simulink model "SVPWM6kHz"  (R2025b)
settings: Solver=VariableStepAuto  StartTime=0.0  StopTime=2  MaxStep=1e-6  RelTol=1e-3  EnableMultiTasking=on
undefined symbols (not defined in the file): Down, SVPWM6kHz, Up
libraries: nesl_utility x11, ee_lib x7, fl_lib x6, peripheralslib x3, prociolib x3, slpidlib x2, eeTransforms x2, simulink x1, eeSinusoidalMeasurement x1
settings Model: ExtModeTrigDuration=8  Creator=18483  LastModifiedBy=18483
settings OptimizationCC: DefaultParameterBehavior=Inlined  DefaultUnderspecifiedDataType=single  EnhancedBackFolding=on  PassReuseOutputArgsAs=Individual arguments  MaxStackSize=1024  OptimizeBlockOrder=speed  DifferentSizesBufferReuse=on  OptimizationCustomize=off  EfficientTunableParamExpr=on
settings DebuggingCC: ParameterTunabilityLossMsg=error
settings HardwareCC: ProdBitPerChar=16.0  ProdBitPerInt=16.0  ProdBitPerPointer=32.0  ProdBitPerSizeT=32.0  ProdBitPerPtrDiffT=32.0  ProdLargestAtomicInteger=Integer  ProdLargestAtomicFloat=None  ProdWordSize=16.0  ProdLongLongMode=on  ProdHWDeviceType=Texas Instruments->C2000  HardwareBoardFeatureSet=SoCBlockset
settings SFSimCC: MATLABDynamicMemAlloc=off
settings RTWCC: SystemTargetFile=ert.tlc  HardwareBoard=TI Delfino F28379D LaunchPad  TemplateMakefile=ert_default_tmf  Toolchain=Texas Instruments Code Composer Studio (C2000)  CodeProfilingSaveOptions=MetricsOnly  Description=Embedded Coder
settings CodeAppCC: ForceParamTrailComments=on  IgnoreCustomStorageClasses=off  OperatorAnnotations=on  SimulinkDataObjDesc=on  SFDataObjDesc=on  InsertBlockDesc=on
settings ERTTargetCC: ExtModeTransport=4.0  ExtModeStaticAlloc=on  ExtModeAutomaticAllocSize=off  ExtModeStaticAllocSize=10000.0  ExtModeMexFile=ext_xcp  ExtModeIntrfLevel=Level2 - Open  CodeReplacementLibrary=TI C28x

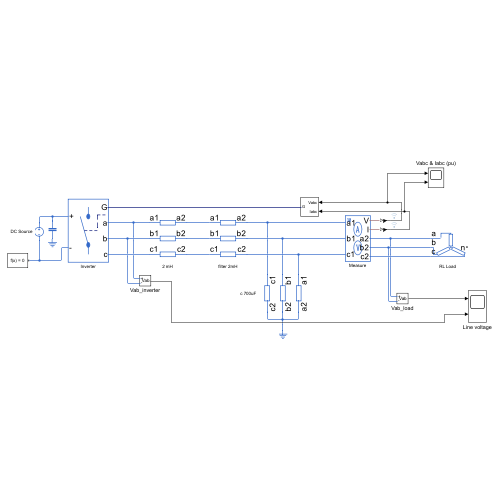
[thumbnail: Simulink's stored preview of the top-level diagram]
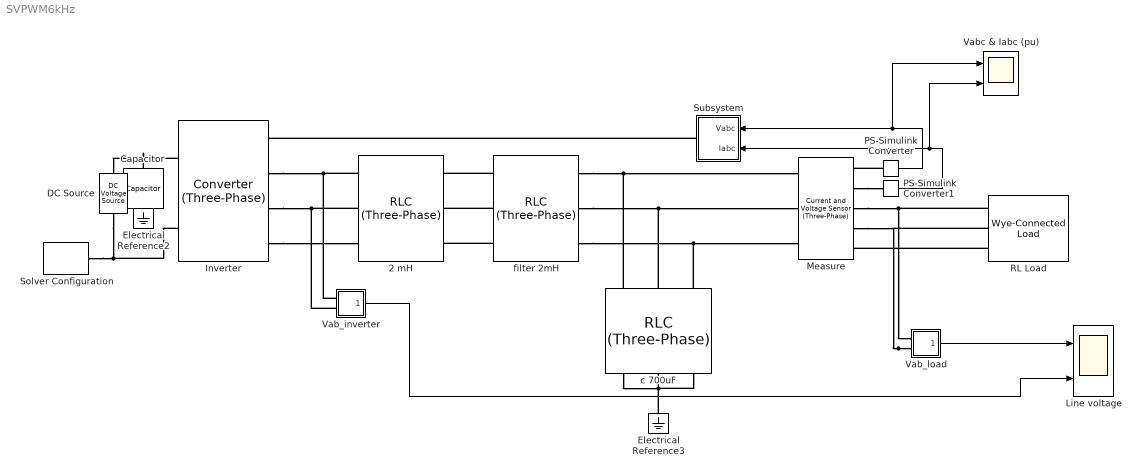
== system SVPWM6kHz ==
  2 mH : ee_lib/Passive/RLC Assemblies/RLC (Three-Phase)  port_option=ee.enum.threePhasePort.expanded  component_structure=ee.enum.rlc.structure.L  R=1 Ohm  L=2 mH  C=1 F  R_parasitic=1e-6 Ohm  G_parasitic=1e-6 1/Ohm  IL_specify=on  IL_priority=High  IL=[0, 0, 0] A  IL_nominal_specify=off  IL_nominal_value=1  IL_nominal_unit=A  VC_specify=on  VC_priority=High  VC=[0, 0, 0] V  VC_nominal_specify=off  VC_nominal_value=1  VC_nominal_unit=V
      settings: InternalSimscapePortConfiguration="{\"Bottom\":[],\"Left\":[{\"id\":\"a1\",\"label\":\"a1\",\"type\":\"foundation.electrical.electrical\"},{\"id\":\"b1\",\"label\":\"b1\",\"type\":\"foundation.electrical.electrical\"},{\"id\":\"c1\",\"label\":\"c1\",\"type\":\"foundation.electrical.electrical\"}],\"Right\":[{\"id\":\"a2\",\"label\":\"a2\",\"type\":\"foundation.electrical.electrical\"},{\"id\":\"b2\",\"label\":\"b2\",\"type\":\"foundation.electrical.electrical\"},{\"id\":\"c2\",\"label\":\"c2\",\"type\":\"foundation.electrical.electrical\"}],\"Top\":[]}"
  Capacitor : fl_lib/Electrical/Electrical Elements/Capacitor  c=1000 uF  r=1e-6 Ohm  g=0 1/Ohm  i_specify=off  i_priority=None  i=0 A  i_nominal_specify=off  i_nominal_value=1  i_nominal_unit=A  v_specify=off  v_priority=None  v=0 V  v_nominal_specify=off  v_nominal_value=1  v_nominal_unit=V  vc_specify=off  vc_priority=High  vc=0 V  vc_nominal_specify=off  vc_nominal_value=1  vc_nominal_unit=V
  DC Source : fl_lib/Electrical/Electrical Sources/DC Voltage Source  v0=60 V
  Electrical Reference2 : fl_lib/Electrical/Electrical Elements/Electrical Reference
  Electrical Reference3 : fl_lib/Electrical/Electrical Elements/Electrical Reference
  Inverter : ee_lib/Semiconductors & Converters/Converters/Converter (Three-Phase)  port_option=ee.enum.threePhasePort.expanded  fidelity_option=ee.enum.converters.fidelity.detailed  device_type=ee.enum.converters.switchingdevice.igbt  showThermalPort=false  K=0  Vth=0.5 V  Vgt=1e-3 V  Vgt_off=-1 V  Ih=1e-4 A  Vf=0.8 V  Ron=1e-3 Ohm  Rds=0.001 Ohm  Goff=1e-5 1/Ohm  Eon_scalar=22.86e-3 J  Eoff_scalar=17.14e-3 J  Eoff_natural_commutation=10e-3 J  Voff=300 V  Iout_scalar=600 A  onCurrentMeasDelay=0 s  useCurrentFromPreviousCycle=false  useVoltageFromPreviousCycle=false  diode_param=ee.enum.converters.protectiondiode.nodynamics  diode_Vf=0.8 V  diode_Ron=0.001 Ohm  diode_Goff=1e-5 1/Ohm  diode_C=50 nF  diode_iRM=-235 A  diode_iF=300 A  diode_idot=-50 A/us  diode_trr_param=ee.enum.converters.diodetrr.trr_factor  diode_trr_factor=3  diode_trr=15 us  diode_Qrr=1.5e+3 s*uA  diode_rec_loss_model=ee.enum.diode.reverseRecoveryModel.fixed  diode_ErecVal=0 J  diode_scaleWithIandV=false  diode_ErecMat=zeros(2, 3) J  diode_TjrecVec=[298.15, 398.15] K  diode_IfrecVec=[.1, 1, 10] A  diode_IrecVal=10 A  diode_VrecVal=10 V  diode_tFilter=1 / 1000 / 100 s  thermal_network_parameterization=ee.enum.thermalNetworkTopology.external  Rth=[.08, .5] K/W  Rth_Cauer=[.08, .1, .5] K/W  Rth_Foster=[.08, .14, .22, .16] K/W  thermal_mass_parameterization=ee.enum.thermalNetwork.timeconstant  thermal_mass=[.01, .5] J/K  thermal_mass_Cauer=[.01, .1, .5] J/K  thermal_mass_Foster=[.001, .005, .05, .5] J/K  thermal_time_constant=[.001, .2] s  thermal_time_constant_Cauer=[.001, .1, .2] s  thermal_time_constant_Foster=[7e-05, .0007, .01, .08] s  thermal_mass_initial_temperatures=[25, 25] degC  thermal_mass_initial_temperatures_Cauer=[25, 25, 25] degC  junction_thermal_mass=0.01 J/K  Tvec_initial_Foster=[25, 25, 25, 25] degC  snubber_type=ee.enum.converters.snubber.exclude  Cs=1e-7 F  Rs=0.1 Ohm  Vce_loss=[0, 150, 300] V
      settings: InternalSimscapePortConfiguration="{\"Bottom\":[],\"Left\":[{\"id\":\"G\",\"label\":\"G\",\"type\":\"foundation.electrical.twelve_phase\"},{\"id\":\"a\",\"label\":\"a\",\"type\":\"foundation.electrical.electrical\"},{\"id\":\"b\",\"label\":\"b\",\"type\":\"foundation.electrical.electrical\"},{\"id\":\"c\",\"label\":\"c\",\"type\":\"foundation.electrical.electrical\"}],\"Right\":[{\"id\":\"p\",\"label\":\"+\",\"type\":\"foundation.electrical.electrical\"},{\"id\":\"n\",\"label\":\"-\",\"type\":\"foundation.electrical.electrical\"}],\"Top\":[]}"
  Line voltage : Scope  NumInputPorts=2
      settings: ActiveDisplayYMinimum=-20.789782785559193  ActiveDisplayYMaximum=20.919388792014789
  Measure : ee_lib/Sensors & Transducers/Current and Voltage Sensor (Three-Phase)  vMeasurementType=ee.enum.vmeasurement.lg  outputUnit=1  SRated=5.196152422706632 V*A  VRated=60/sqrt(2) V  I_specify=off  I_priority=None  I=[ 0 0 0 ] A  I_nominal_specify=off  I_nominal_value=1  I_nominal_unit=A  V_specify=off  V_priority=None  V=[ 0 0 0 ] V  V_nominal_specify=off  V_nominal_value=1  V_nominal_unit=V
      settings: InternalSimscapePortConfiguration="{\"Bottom\":[],\"Left\":[{\"id\":\"a1\",\"label\":\"a1\",\"type\":\"foundation.electrical.electrical\"},{\"id\":\"b1\",\"label\":\"b1\",\"type\":\"foundation.electrical.electrical\"},{\"id\":\"c1\",\"label\":\"c1\",\"type\":\"foundation.electrical.electrical\"}],\"Right\":[{\"id\":\"V_output\",\"label\":\"V\",\"type\":\"output\"},{\"id\":\"I_output\",\"label\":\"I\",\"type\":\"output\"},{\"id\":\"a2\",\"label\":\"a2\",\"type\":\"foundation.electrical.electrical\"},{\"id\":\"b2\",\"label\":\"b2\",\"type\":\"foundation.electrical.electrical\"},{\"id\":\"c2\",\"label\":\"c2\",\"type\":\"foundation.electrical.electrical\"}],\"Top\":[]}"
  PS-Simulink Converter : nesl_utility/PS-Simulink Converter  PhysicalDomain=network_engine_domain  SubClassName=ps_output  LeftPortType=input  RightPortType=output  PseudoPeriodic=off  Frequencies=[]  VectorFormat=1-D array  Unit=inherit  AffineConversion=off
  PS-Simulink Converter1 : nesl_utility/PS-Simulink Converter  PhysicalDomain=network_engine_domain  SubClassName=ps_output  LeftPortType=input  RightPortType=output  PseudoPeriodic=off  Frequencies=[]  VectorFormat=1-D array  Unit=inherit  AffineConversion=off
  "RL Load " : ee_lib/Passive/RLC Assemblies/Wye-Connected Load  port_option=ee.enum.threePhasePort.expanded  parameterization=1  component_structure=ee.enum.rlc.structure.SeriesRL  component_structure_PQ=ee.enum.rlc.structure.R  R=685.7142857142857 Ohm  L=2.173457943925234 H  C=1e-6 F  VRated=60 V  FRated=50 Hz  P=50000 W  Qpos=37500 V*A  Qneg=-1000 V*A  R_parasitic=1e-6 Ohm  G_parasitic=1e-6 1/Ohm  R_parasitic_PQ=1e-6 Ohm  G_parasitic_PQ=1e-6 1/Ohm  Vmag0=380 V  Vang0=0 deg  Freq0=50 Hz  IL_specify=on  IL_priority=High  IL=[ 0 0 0 ] A  IL_nominal_specify=off  IL_nominal_value=1  IL_nominal_unit=A  VC_specify=on  VC_priority=High  VC=[ 0 0 0 ] V  VC_nominal_specify=off  VC_nominal_value=1  VC_nominal_unit=V
      settings: InternalSimscapePortConfiguration="{\"Bottom\":[],\"Left\":[{\"id\":\"a\",\"label\":\"a\",\"type\":\"foundation.electrical.electrical\"},{\"id\":\"b\",\"label\":\"b\",\"type\":\"foundation.electrical.electrical\"},{\"id\":\"c\",\"label\":\"c\",\"type\":\"foundation.electrical.electrical\"}],\"Right\":[{\"id\":\"n\",\"label\":\"n\",\"type\":\"foundation.electrical.electrical\"}],\"Top\":[]}"
  Solver Configuration : nesl_utility/Solver Configuration  PhysicalDomain=network_engine_domain  SubClassName=solver  LeftPortType=input  RightPortType=generic  Tones=[]  Harmonics=[]  SimulateNoise=off  Profile=off  UseLocalSampling=off  EnableSwitchedLinearOptims=on  FrequencyDomain=off  UseCCode=off  RelTol=0.001  AbsTol=1e-06  MinStep=1e-09  ToWorkspace=off  RevertToSquareIcSolve=off  NumHomotopyIterations=100  PhasorMode=off  PhasorModeNumHarmonics=1  ConsistencySolver=NEWTON_FTOL  IndexReductionMethod=DerivativeReplacement  DoDC=off  ResidualTolerance=1e-09  ConsistencyTolSource=GLOBAL  ConsistencyAbsTol=0.001  ConsistencyRelTol=0.001  ConsistencyTolFactor=0.001  UseLocalSolver=on  LocalSolverChoice=NE_BACKWARD_EULER_ADVANCER  ResolveIndetEquations=on  FunctionEvalNumThread=1  LocalSolverSampleTime=5e-7  DoFixedCost=off  MaxNonlinIter=3  MaxModeIter=2  ComputeImpulses=off  ImpulseIterations=1  LinearAlgebra=auto  LinearAlgebraNumThread=0  EquationFormulation=NE_TIME_EF  DelaysMemoryBudget=1024  AutomaticFiltering=on  FilteringTimeConstant=0.001  PartitionStorageMethod=AS_NEEDED  PartitionMemoryBudget=1024  PartitionMethod=FAST  MultibodyUseLocalSolver=off  MultibodyLocalSolverChoice=ODE1  MultibodyLocalSolverSampleTime=0.001
  Subsystem : Subsystem
  Vab_inverter : Subsystem  Tag=PoWeRsYsTeMmEaSuReMeNt
  Vab_load : Subsystem  Tag=PoWeRsYsTeMmEaSuReMeNt
  Vabc & Iabc (pu) : Scope  NumInputPorts=2
      settings: ActiveDisplayYMinimum=-0.75930761819082393  ActiveDisplayYMaximum=0.20930609176345122
  c 700uF : ee_lib/Passive/RLC Assemblies/RLC (Three-Phase)  port_option=ee.enum.threePhasePort.expanded  component_structure=ee.enum.rlc.structure.C  R=7.5 Ohm  L=0.0005 H  C=70e-5 F  R_parasitic=1e-6 Ohm  G_parasitic=1e-6 1/Ohm  IL_specify=on  IL_priority=High  IL=[0, 0, 0] A  IL_nominal_specify=off  IL_nominal_value=1  IL_nominal_unit=A  VC_specify=on  VC_priority=High  VC=[0, 0, 0] V  VC_nominal_specify=off  VC_nominal_value=1  VC_nominal_unit=V
      settings: InternalSimscapePortConfiguration="{\"Bottom\":[],\"Left\":[{\"id\":\"a1\",\"label\":\"a1\",\"type\":\"foundation.electrical.electrical\"},{\"id\":\"b1\",\"label\":\"b1\",\"type\":\"foundation.electrical.electrical\"},{\"id\":\"c1\",\"label\":\"c1\",\"type\":\"foundation.electrical.electrical\"}],\"Right\":[{\"id\":\"a2\",\"label\":\"a2\",\"type\":\"foundation.electrical.electrical\"},{\"id\":\"b2\",\"label\":\"b2\",\"type\":\"foundation.electrical.electrical\"},{\"id\":\"c2\",\"label\":\"c2\",\"type\":\"foundation.electrical.electrical\"}],\"Top\":[]}"
  filter 2mH : ee_lib/Passive/RLC Assemblies/RLC (Three-Phase)  port_option=ee.enum.threePhasePort.expanded  component_structure=ee.enum.rlc.structure.L  R=1 Ohm  L=2e-3 H  C=1 F  R_parasitic=1e-6 Ohm  G_parasitic=1e-6 1/Ohm  IL_specify=on  IL_priority=High  IL=[0, 0, 0] A  IL_nominal_specify=off  IL_nominal_value=1  IL_nominal_unit=A  VC_specify=on  VC_priority=High  VC=[0, 0, 0] V  VC_nominal_specify=off  VC_nominal_value=1  VC_nominal_unit=V
      settings: InternalSimscapePortConfiguration="{\"Bottom\":[],\"Left\":[{\"id\":\"a1\",\"label\":\"a1\",\"type\":\"foundation.electrical.electrical\"},{\"id\":\"b1\",\"label\":\"b1\",\"type\":\"foundation.electrical.electrical\"},{\"id\":\"c1\",\"label\":\"c1\",\"type\":\"foundation.electrical.electrical\"}],\"Right\":[{\"id\":\"a2\",\"label\":\"a2\",\"type\":\"foundation.electrical.electrical\"},{\"id\":\"b2\",\"label\":\"b2\",\"type\":\"foundation.electrical.electrical\"},{\"id\":\"c2\",\"label\":\"c2\",\"type\":\"foundation.electrical.electrical\"}],\"Top\":[]}"
  wires:
  Vab_load/1(Vab) -> Line voltage/1
  PS-Simulink Converter1/1 -> Vabc & Iabc (pu)/2, Subsystem/2(Iabc)
  PS-Simulink Converter/1 -> Vabc & Iabc (pu)/1, Subsystem/1(Vabc)
  Vab_inverter/1(Vab) -> Line voltage/2
  connections:
  Measure/RConn3 -- "RL Load "/LConn1 -- Vab_load/LConn1
  Solver Configuration/RConn1 -- DC Source/RConn1 -- Inverter/RConn2
  2 mH/LConn1 -- Inverter/LConn2 -- Vab_inverter/LConn1
  filter 2mH/LConn1 -- 2 mH/RConn1
  filter 2mH/LConn3 -- 2 mH/RConn3
  filter 2mH/LConn2 -- 2 mH/RConn2
  2 mH/LConn2 -- Inverter/LConn3 -- Vab_inverter/LConn2
  Vab_load/LConn2 -- "RL Load "/LConn2 -- Measure/RConn4
  "RL Load "/LConn3 -- Measure/RConn5
  Measure/RConn2 -- PS-Simulink Converter1/LConn1
  PS-Simulink Converter/LConn1 -- Measure/RConn1
  Inverter/RConn1 -- DC Source/LConn1 -- Capacitor/LConn1
  Inverter/LConn4 -- 2 mH/LConn3
  filter 2mH/RConn1 -- Measure/LConn1 -- c 700uF/LConn3
  filter 2mH/RConn2 -- Measure/LConn2 -- c 700uF/LConn2
  filter 2mH/RConn3 -- Measure/LConn3 -- c 700uF/LConn1
  c 700uF/RConn3 -- c 700uF/RConn1 -- Electrical Reference3/LConn1 -- c 700uF/RConn2
  Subsystem/RConn1 -- Inverter/LConn1
  Electrical Reference2/LConn1 -- Capacitor/RConn1

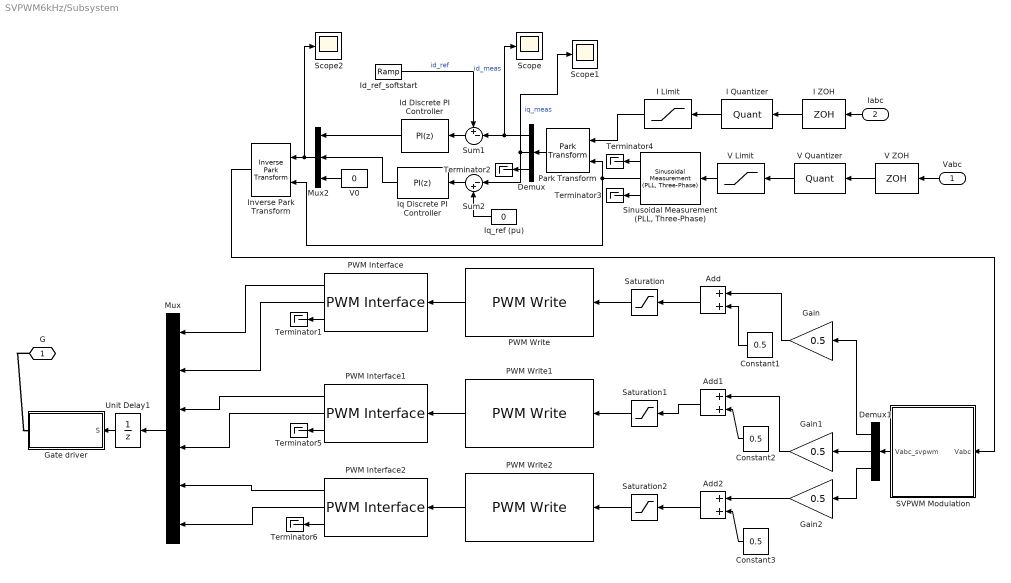
== system SVPWM6kHz/Subsystem ==
  Vabc : Inport
  Iabc : Inport  Port=2
  Add : Sum
  Add1 : Sum
  Add2 : Sum
  Constant1 : Constant  Value=0.5
  Constant2 : Constant  Value=0.5
  Constant3 : Constant  Value=0.5
  Demux : Demux  Outputs=3
  Demux1 : Demux  Outputs=3
  Gain : Gain  Gain=0.5
  Gain1 : Gain  Gain=0.5
  Gain2 : Gain  Gain=0.5
  Gate driver : Subsystem
  I Limit : Saturate  UpperLimit=3  LowerLimit=-3
  I Quantizer : Quantizer  QuantizationInterval=4/4095
  I ZOH : ZeroOrderHold  SampleTime=0.0001666666666666667
  Id Discrete PI Controller : slpidlib/PID Controller  Controller=PI  Form=Parallel  TimeDomain=Discrete-time  UseExternalTs=off  SampleTime=0.0001666666666666667  IntegratorMethod=Forward Euler  FilterMethod=Forward Euler  ControllerParametersSource=internal  P=0.2  I=64  UseKiTs=off  D=0  UseExternalDerivativeSource=off  N=100  UseFilter=on  TunerSelectOption=Transfer Function Based (PID Tuner App)  InitialConditionSource=internal  InitialConditionForIntegrator=0  InitialConditionForFilter=0  DifferentiatorICPrevScaledInput=0  ExternalReset=none  TrackingMode=off  Kt=1  LimitOutput=on  SatLimitsSource=internal  UpperSaturationLimit=0.65  LowerSaturationLimit=-0.65  LinearizeAsGain=on  AntiWindupMode=clamping  Kb=1  LimitIntegrator=off  UpperIntegratorSaturationLimit=inf  LowerIntegratorSaturationLimit=-inf  POutMin=[]  POutMax=[]  IOutMin=[]  IOutMax=[]  DOutMin=[]  DOutMax=[]  NOutMin=[]  NOutMax=[]  SumOutMin=[]  SumOutMax=[]  SaturationOutMin=[]  SaturationOutMax=[]  PParamMin=[]  PParamMax=[]  IParamMin=[]  IParamMax=[]  DParamMin=[]  DParamMax=[]  NParamMin=[]  NParamMax=[]  KbParamMin=[]  KbParamMax=[]  KtParamMin=[]  KtParamMax=[]  KbOutMin=[]  KbOutMax=[]  KtOutMin=[]  KtOutMax=[]  IntegratorOutMin=[]  IntegratorOutMax=[]  FilterOutMin=[]  FilterOutMax=[]  SumI1OutMin=[]  SumI1OutMax=[]  SumI2OutMin=[]  SumI2OutMax=[]  SumI3OutMin=[]  SumI3OutMax=[]  SumI4OutMin=[]  SumI4OutMax=[]  SumDOutMin=[]  SumDOutMax=[]  DifferentiatorOutMin=[]  DifferentiatorOutMax=[]  FilterDiffOutCoefMin=[]  FilterDiffOutCoefMax=[]  ReciprocalOutMin=[]  ReciprocalOutMax=[]  SumDenOutMin=[]  SumDenOutMax=[]  SumNumOutMin=[]  SumNumOutMax=[]  DivideOutMin=[]  DivideOutMax=[]  UdiffTsProdOutMin=[]  UdiffTsProdOutMax=[]  NTsProdOutMin=[]  NTsProdOutMax=[]  UintegralTsProdOutMin=[]  UintegralTsProdOutMax=[]  UngainTsProdOutMin=[]  UngainTsProdOutMax=[]  ClampingZeroOutDataTypeStr=Inherit: Inherit via back propagation  ClampingZeroOutMin=[]  ClampingZeroOutMax=[]  FilterDenConstantOutDataTypeStr=Inherit: Inherit via back propagation  FilterDenConstantOutMin=[]  FilterDenConstantOutMax=[]  PCopyOutDataTypeStr=Inherit: Inherit via back propagation  PCopyOutMin=[]  PCopyOutMax=[]  NCopyOutDataTypeStr=Inherit: Inherit via back propagation  NCopyOutMin=[]  NCopyOutMax=[]  IntegratorContinuousStateAttributes=''  IntegratorStateMustResolveToSignalObject=off  IntegratorRTWStateStorageClass=Auto  FilterContinuousStateAttributes=''  FilterStateMustResolveToSignalObject=off  FilterRTWStateStorageClass=Auto  ParallelPVariant=InternalParameters  IdealPVariant=Disabled  IVariant=InternalParameters  DVariant=Disabled  IntegratorVariant=Discrete  SatVariant=Enabled  AWVariant=DiscClampingParallel  PCopyVariant=Disabled  TRVariant=Disabled  FdbkBlocksVariant=Forward  IdealPFdbkVariant=Disabled  SatFdbkVariant=Disabled  DerivativeFilterVariant=Disabled  NVariant=Disabled  NCopyVariant=Disabled_SignalSpec  FilterICVariant=Disabled  IntegratorICVariant=InternalICs  ExternalResetVariant=Disabled  TRSumVariant=Passthrough  SumFdbkVariant=Disabled  SumVariant=Sum_PI  TsampFilterVariant=InternalTs  TsampNgainVariant=Passthrough  TsampIntegralVariant=Disabled_SignalSpec  ExternalSaturationOutDataTypeStr=Inherit: Same as second input  DerivativeSourceVariant=Disabled  PreIntVariant=InternalPreInt
  Id_ref_softstart : simulink/Sources/Ramp  slope=0  start=0  InitialOutput=0.076
  Inverse Park Transform : eeTransforms/Inverse Park Transform  AxisAlignment=Q-axis  PowerInvariant=off
      link override b: Expr=sin(u(4)+Offset-2.0943951023931953)*u(1) + cos(u(4)+Offset-2.0943951023931953)*u(2) + K1*u(3)
      link override c: Expr=sin(u(4)+Offset+2.0943951023931953)*u(1) + cos(u(4)+Offset+2.0943951023931953)*u(2) + K1*u(3)
  Iq Discrete PI Controller : slpidlib/PID Controller  Controller=PI  Form=Parallel  TimeDomain=Discrete-time  UseExternalTs=off  SampleTime=0.0001666666666666667  IntegratorMethod=Forward Euler  FilterMethod=Forward Euler  ControllerParametersSource=internal  P=0.2  I=64  UseKiTs=off  D=0  UseExternalDerivativeSource=off  N=100  UseFilter=on  TunerSelectOption=Transfer Function Based (PID Tuner App)  InitialConditionSource=internal  InitialConditionForIntegrator=0  InitialConditionForFilter=0  DifferentiatorICPrevScaledInput=0  ExternalReset=none  TrackingMode=off  Kt=1  LimitOutput=on  SatLimitsSource=internal  UpperSaturationLimit=0.65  LowerSaturationLimit=-0.65  LinearizeAsGain=on  AntiWindupMode=clamping  Kb=1  LimitIntegrator=off  UpperIntegratorSaturationLimit=inf  LowerIntegratorSaturationLimit=-inf  POutMin=[]  POutMax=[]  IOutMin=[]  IOutMax=[]  DOutMin=[]  DOutMax=[]  NOutMin=[]  NOutMax=[]  SumOutMin=[]  SumOutMax=[]  SaturationOutMin=[]  SaturationOutMax=[]  PParamMin=[]  PParamMax=[]  IParamMin=[]  IParamMax=[]  DParamMin=[]  DParamMax=[]  NParamMin=[]  NParamMax=[]  KbParamMin=[]  KbParamMax=[]  KtParamMin=[]  KtParamMax=[]  KbOutMin=[]  KbOutMax=[]  KtOutMin=[]  KtOutMax=[]  IntegratorOutMin=[]  IntegratorOutMax=[]  FilterOutMin=[]  FilterOutMax=[]  SumI1OutMin=[]  SumI1OutMax=[]  SumI2OutMin=[]  SumI2OutMax=[]  SumI3OutMin=[]  SumI3OutMax=[]  SumI4OutMin=[]  SumI4OutMax=[]  SumDOutMin=[]  SumDOutMax=[]  DifferentiatorOutMin=[]  DifferentiatorOutMax=[]  FilterDiffOutCoefMin=[]  FilterDiffOutCoefMax=[]  ReciprocalOutMin=[]  ReciprocalOutMax=[]  SumDenOutMin=[]  SumDenOutMax=[]  SumNumOutMin=[]  SumNumOutMax=[]  DivideOutMin=[]  DivideOutMax=[]  UdiffTsProdOutMin=[]  UdiffTsProdOutMax=[]  NTsProdOutMin=[]  NTsProdOutMax=[]  UintegralTsProdOutMin=[]  UintegralTsProdOutMax=[]  UngainTsProdOutMin=[]  UngainTsProdOutMax=[]  ClampingZeroOutDataTypeStr=Inherit: Inherit via back propagation  ClampingZeroOutMin=[]  ClampingZeroOutMax=[]  FilterDenConstantOutDataTypeStr=Inherit: Inherit via back propagation  FilterDenConstantOutMin=[]  FilterDenConstantOutMax=[]  PCopyOutDataTypeStr=Inherit: Inherit via back propagation  PCopyOutMin=[]  PCopyOutMax=[]  NCopyOutDataTypeStr=Inherit: Inherit via back propagation  NCopyOutMin=[]  NCopyOutMax=[]  IntegratorContinuousStateAttributes=''  IntegratorStateMustResolveToSignalObject=off  IntegratorRTWStateStorageClass=Auto  FilterContinuousStateAttributes=''  FilterStateMustResolveToSignalObject=off  FilterRTWStateStorageClass=Auto  ParallelPVariant=InternalParameters  IdealPVariant=Disabled  IVariant=InternalParameters  DVariant=Disabled  IntegratorVariant=Discrete  SatVariant=Enabled  AWVariant=DiscClampingParallel  PCopyVariant=Disabled  TRVariant=Disabled  FdbkBlocksVariant=Forward  IdealPFdbkVariant=Disabled  SatFdbkVariant=Disabled  DerivativeFilterVariant=Disabled  NVariant=Disabled  NCopyVariant=Disabled_SignalSpec  FilterICVariant=Disabled  IntegratorICVariant=InternalICs  ExternalResetVariant=Disabled  TRSumVariant=Passthrough  SumFdbkVariant=Disabled  SumVariant=Sum_PI  TsampFilterVariant=InternalTs  TsampNgainVariant=Passthrough  TsampIntegralVariant=Disabled_SignalSpec  ExternalSaturationOutDataTypeStr=Inherit: Same as second input  DerivativeSourceVariant=Disabled  PreIntVariant=InternalPreInt
  Iq_ref (pu) : Constant  Value=0
  Mux : Mux  Inputs=6
  Mux2 : Mux  Inputs=3
  PWM Interface : peripheralslib/PWM Interface  Period=0.0001666666666666667  OutSigMode=Switching  CounterMode=Up-Down  GenCompPWM=on  DeadTimeTopPWM=1e-6  DeadTimeBottomPWM=1e-6  EventCondition2=End of PWM period  DataType=double  PWMAtStartPeriod=High  PWMAtMidPeriod=NoChange  PWMAtCMP1=Low  PWMAtCMP1UpCnt=Low  PWMAtCMP1DwnCnt=High  PWMAtCMP2=NoChange  PWMAtCMP2UpCnt=NoChange  PWMAtCMP2DwnCnt=NoChange  OutCountDir=off  PhaseOffset=0  EventType=ADC start  EventCondition1=End of PWM period  NumADCSOCToWait=1st event  NumADCSOCReplica=1  InterruptCond=End of PWM period  IntLatency=0  NumInterruptToWait=1st event
      settings: LibrarySourceBlock=c2btestbenchlib/PWM Interface  SamplingMode=End of PWM period
  PWM Interface1 : peripheralslib/PWM Interface  Period=0.0001666666666666667  OutSigMode=Switching  CounterMode=Up-Down  GenCompPWM=on  DeadTimeTopPWM=1e-6  DeadTimeBottomPWM=1e-6  EventCondition2=End of PWM period  DataType=double  PWMAtStartPeriod=High  PWMAtMidPeriod=NoChange  PWMAtCMP1=Low  PWMAtCMP1UpCnt=Low  PWMAtCMP1DwnCnt=High  PWMAtCMP2=NoChange  PWMAtCMP2UpCnt=NoChange  PWMAtCMP2DwnCnt=NoChange  OutCountDir=off  PhaseOffset=0  EventType=ADC start  EventCondition1=End of PWM period  NumADCSOCToWait=1st event  NumADCSOCReplica=1  InterruptCond=End of PWM period  IntLatency=0  NumInterruptToWait=1st event
      settings: LibrarySourceBlock=c2btestbenchlib/PWM Interface  SamplingMode=End of PWM period
  PWM Interface2 : peripheralslib/PWM Interface  Period=0.0001666666666666667  OutSigMode=Switching  CounterMode=Up-Down  GenCompPWM=on  DeadTimeTopPWM=1e-6  DeadTimeBottomPWM=1e-6  EventCondition2=End of PWM period  DataType=double  PWMAtStartPeriod=High  PWMAtMidPeriod=NoChange  PWMAtCMP1=Low  PWMAtCMP1UpCnt=Low  PWMAtCMP1DwnCnt=High  PWMAtCMP2=NoChange  PWMAtCMP2UpCnt=NoChange  PWMAtCMP2DwnCnt=NoChange  OutCountDir=off  PhaseOffset=0  EventType=ADC start  EventCondition1=End of PWM period  NumADCSOCToWait=1st event  NumADCSOCReplica=1  InterruptCond=End of PWM period  IntLatency=0  NumInterruptToWait=1st event
      settings: LibrarySourceBlock=c2btestbenchlib/PWM Interface  SamplingMode=End of PWM period
  PWM Write : prociolib/PWM Write  ShowPeriodInp=off  ShowPhaseInp=off  PeripheralConfigBtnCtrl=0  BlockSID=SVPWM6kHz:349
  PWM Write1 : prociolib/PWM Write  ShowPeriodInp=off  ShowPhaseInp=off  PeripheralConfigBtnCtrl=0  BlockSID=SVPWM6kHz:350
  PWM Write2 : prociolib/PWM Write  ShowPeriodInp=off  ShowPhaseInp=off  PeripheralConfigBtnCtrl=0  BlockSID=SVPWM6kHz:351
  Park Transform : eeTransforms/Park Transform  AxisAlignment=Q-axis  PowerInvariant=off
      link override d: Expr=sin(u(4)+Offset)*u(1) + sin(u(4)+Offset-2.0943951023931953)*u(2) + sin(u(4)+Offset+2.0943951023931953)*u(3)
      link override q: Expr=cos(u(4)+Offset)*u(1) + cos(u(4)+Offset-2.0943951023931953)*u(2) + cos(u(4)+Offset+2.0943951023931953)*u(3)
  SVPWM Modulation : Subsystem
  Saturation : Saturate  UpperLimit=0.95  LowerLimit=0.05
  Saturation1 : Saturate  UpperLimit=0.95  LowerLimit=0.05
  Saturation2 : Saturate  UpperLimit=0.95  LowerLimit=0.05
  Scope : Scope
      settings: ActiveDisplayYMinimum=-1  ActiveDisplayYMaximum=1  DataLoggingVariableName=ScopeData2
  Scope1 : Scope
      settings: ActiveDisplayYMinimum=-1  ActiveDisplayYMaximum=1  DataLoggingVariableName=ScopeData3
  Scope2 : Scope
      settings: ActiveDisplayYMinimum=-0.0129121107959027  ActiveDisplayYMaximum=0.1161479259377293  DataLoggingVariableName=ScopeData4
  "Sinusoidal Measurement (PLL, Three-Phase)" : eeSinusoidalMeasurement/Sinusoidal Measurement (PLL, Three-Phase)  Kp_LF=0  Ki_LF=0  F0=50  Theta0=0  Ts=0.0001666666666666667
      link override Angle/Integrator with Wrapped State (Discrete or Continuous): WrappedStateUpperValue=6.283185307179586
      link override Gain1: Gain=0.15915494309189535
      link override PI/Constant: Value=314.1592653589793
      link override Park Transform/d: Expr=sin(u(4)+Offset)*u(1) + sin(u(4)+Offset-2.0943951023931953)*u(2) + sin(u(4)+Offset+2.0943951023931953)*u(3)
      link override Park Transform/q: Expr=cos(u(4)+Offset)*u(1) + cos(u(4)+Offset-2.0943951023931953)*u(2) + cos(u(4)+Offset+2.0943951023931953)*u(3)
  Sum1 : Sum  Inputs=+-|  InputSameDT=on  SaturateOnIntegerOverflow=on  OutDataTypeStr=Inherit: Same as first input
  Sum2 : Sum  Inputs=|-+  InputSameDT=on  SaturateOnIntegerOverflow=on  OutDataTypeStr=Inherit: Same as first input
  Terminator{1..6} (6 alike) : Terminator
      Terminator1 settings: InputPortMessageModes=m
      Terminator5 settings: InputPortMessageModes=m
      Terminator6 settings: InputPortMessageModes=m
  Unit Delay1 : UnitDelay  SampleTime=-1  HasFrameUpgradeWarning=on
  V Limit : Saturate  UpperLimit=1.2  LowerLimit=-1.2
  V Quantizer : Quantizer  QuantizationInterval=4/4095
  V ZOH : ZeroOrderHold  SampleTime=0.0001666666666666667
  V0 : Constant  Value=0
  G : PMIOPort  Side=Right
  wires:
  Iq Discrete PI Controller/1 -> Mux2/2
  Iq_ref (pu)/1 -> Sum2/2
  Demux/3 -> Terminator2/1
  Park Transform/1 -> Demux/1
  Sum1/1 -> Id Discrete PI Controller/1
  Sum2/1 -> Iq Discrete PI Controller/1
  Mux2/1 -> Scope2/1, Inverse Park Transform/1
  Demux/1 -> Scope/1, Sum1/2  "id_meas"
  "Sinusoidal Measurement (PLL, Three-Phase)"/2 -> Park Transform/2, Inverse Park Transform/2
  Demux/2 -> Sum2/1, Scope1/1  "iq_meas"
  Id Discrete PI Controller/1 -> Mux2/1
  V0/1 -> Mux2/3
  "Sinusoidal Measurement (PLL, Three-Phase)"/3 -> Terminator3/1
  Id_ref_softstart/1 -> Sum1/1  "id_ref"
  V Limit/1 -> "Sinusoidal Measurement (PLL, Three-Phase)"/1
  I Limit/1 -> Park Transform/1
  PWM Interface2/2 -> Mux/6
  Constant1/1 -> Add/2
  Demux1/3 -> Gain2/1
  Add2/1 -> Saturation2/1
  PWM Interface2/1 -> Mux/5
  Saturation2/1 -> PWM Write2/1
  PWM Interface/2 -> Mux/2
  PWM Write2/1 -> PWM Interface2/1
  Demux1/1 -> Gain/1
  Add/1 -> Saturation/1
  Mux/1 -> Unit Delay1/1
  PWM Interface1/2 -> Mux/4
  Constant3/1 -> Add2/2
  PWM Interface/1 -> Mux/1
  Unit Delay1/1 -> Gate driver/1(S)
  Gain/1 -> Add/1
  Saturation/1 -> PWM Write/1
  PWM Interface1/1 -> Mux/3
  PWM Write1/1 -> PWM Interface1/1
  PWM Interface2/3 -> Terminator6/1
  Saturation1/1 -> PWM Write1/1
  PWM Interface/3 -> Terminator1/1
  Gain2/1 -> Add2/1
  PWM Write/1 -> PWM Interface/1
  Add1/1 -> Saturation1/1
  Inverse Park Transform/1 -> SVPWM Modulation/1(Vabc)
  Gain1/1 -> Add1/1
  SVPWM Modulation/1(Vabc_svpwm) -> Demux1/1
  Demux1/2 -> Gain1/1
  PWM Interface1/3 -> Terminator5/1
  Constant2/1 -> Add1/2
  Iabc/1 -> I ZOH/1
  V Quantizer/1 -> V Limit/1
  V ZOH/1 -> V Quantizer/1
  I ZOH/1 -> I Quantizer/1
  I Quantizer/1 -> I Limit/1
  Vabc/1 -> V ZOH/1
  "Sinusoidal Measurement (PLL, Three-Phase)"/1 -> Terminator4/1
  connections:
  G/RConn1 -- Gate driver/RConn1

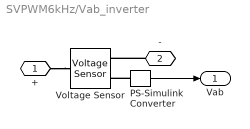
== system SVPWM6kHz/Vab_inverter ==
  PS-Simulink Converter : nesl_utility/PS-Simulink Converter  PhysicalDomain=network_engine_domain  SubClassName=ps_output  LeftPortType=input  RightPortType=output  PseudoPeriodic=off  Frequencies=[]  VectorFormat=1-D array  Unit=V  AffineConversion=off
  Voltage Sensor : fl_lib/Electrical/Electrical Sensors/Voltage Sensor
  + : PMIOPort  Side=Left
  - : PMIOPort  Port=2  Side=Left
  Vab : Outport
  wires:
  PS-Simulink Converter/1 -> Vab/1
  connections:
  +/RConn1 -- Voltage Sensor/LConn1
  -/RConn1 -- Voltage Sensor/RConn2
  PS-Simulink Converter/LConn1 -- Voltage Sensor/RConn1

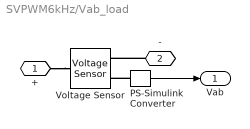
== system SVPWM6kHz/Vab_load ==
  PS-Simulink Converter : nesl_utility/PS-Simulink Converter  PhysicalDomain=network_engine_domain  SubClassName=ps_output  LeftPortType=input  RightPortType=output  PseudoPeriodic=off  Frequencies=[]  VectorFormat=1-D array  Unit=V  AffineConversion=off
  Voltage Sensor : fl_lib/Electrical/Electrical Sensors/Voltage Sensor
  + : PMIOPort  Side=Left
  - : PMIOPort  Port=2  Side=Left
  Vab : Outport
  wires:
  PS-Simulink Converter/1 -> Vab/1
  connections:
  PS-Simulink Converter/LConn1 -- Voltage Sensor/RConn1
  -/RConn1 -- Voltage Sensor/RConn2
  +/RConn1 -- Voltage Sensor/LConn1

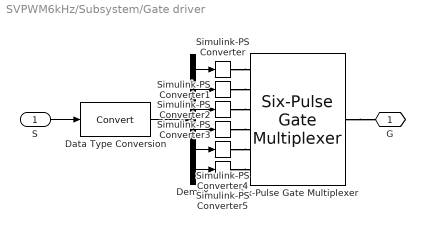
== system SVPWM6kHz/Subsystem/Gate driver ==
  S : Inport
  Data Type Conversion : DataTypeConversion  SaturateOnIntegerOverflow=off  RndMeth=Floor
  Demux : Demux  Outputs=6
  Simulink-PS Converter{,1..5} (6 alike) : nesl_utility/Simulink-PS Converter  PhysicalDomain=network_engine_domain  SubClassName=ps_input  LeftPortType=input  RightPortType=output  PseudoPeriodic=off  Frequencies=[]  NoiseDistribution=none  NoiseParameters=[]  Unit=1  AffineConversion=off  FilteringAndDerivatives=provide  SimscapeFilterOrder=1  InputFilterTimeConstant=0.001  UdotUserProvided=0
  Six-Pulse Gate Multiplexer : ee_lib/Semiconductors & Converters/Converters/Six-Pulse Gate Multiplexer  port_option=ee.enum.controlport.ps
  G : PMIOPort  Side=Right
  wires:
  Demux/5 -> Simulink-PS Converter4/1
  Demux/3 -> Simulink-PS Converter2/1
  Data Type Conversion/1 -> Demux/1
  Demux/4 -> Simulink-PS Converter3/1
  Demux/6 -> Simulink-PS Converter5/1
  Demux/2 -> Simulink-PS Converter1/1
  Demux/1 -> Simulink-PS Converter/1
  S/1 -> Data Type Conversion/1
  connections:
  Simulink-PS Converter4/RConn1 -- Six-Pulse Gate Multiplexer/LConn5
  Simulink-PS Converter2/RConn1 -- Six-Pulse Gate Multiplexer/LConn3
  Simulink-PS Converter/RConn1 -- Six-Pulse Gate Multiplexer/LConn1
  Simulink-PS Converter5/RConn1 -- Six-Pulse Gate Multiplexer/LConn6
  Simulink-PS Converter1/RConn1 -- Six-Pulse Gate Multiplexer/LConn2
  Simulink-PS Converter3/RConn1 -- Six-Pulse Gate Multiplexer/LConn4
  Six-Pulse Gate Multiplexer/RConn1 -- G/RConn1

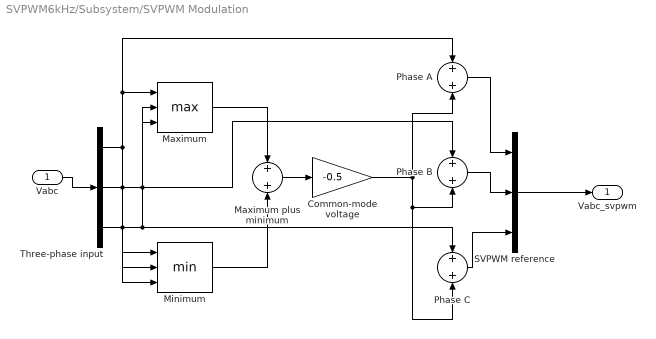
== system SVPWM6kHz/Subsystem/SVPWM Modulation ==
  Vabc : Inport
  Common-mode voltage : Gain  Gain=-0.5
  Maximum : MinMax  Function=max  Inputs=3
  Maximum plus minimum : Sum
  Minimum : MinMax  Inputs=3
  Phase A : Sum
  Phase B : Sum
  Phase C : Sum
  SVPWM reference : Mux  Inputs=3
  Three-phase input : Demux  Outputs=3
  Vabc_svpwm : Outport
  wires:
  Vabc/1 -> Three-phase input/1
  Three-phase input/1 -> Maximum/1, Phase A/1, Minimum/1
  Three-phase input/2 -> Maximum/2, Phase B/1, Minimum/2
  Three-phase input/3 -> Maximum/3, Phase C/1, Minimum/3
  Maximum/1 -> Maximum plus minimum/1
  Minimum/1 -> Maximum plus minimum/2
  Maximum plus minimum/1 -> Common-mode voltage/1
  Common-mode voltage/1 -> Phase B/2, Phase C/2, Phase A/2
  Phase A/1 -> SVPWM reference/1
  Phase B/1 -> SVPWM reference/2
  Phase C/1 -> SVPWM reference/3
  SVPWM reference/1 -> Vabc_svpwm/1
